simulink model "Simscape_Model"  (R2025b)
settings: Solver=ode15s  StartTime=0.0  StopTime=20  RelTol=1e-3
undefined symbols (not defined in the file): c1, c2, g, k1, k2, kt1, kt2, L1, L2, M1, m1, M2, m2, v1_0, v2_0, X, x1_0, x2_0, Y, Z
libraries: sm_lib x18, nesl_utility x9
settings Model: Creator=Utente  LastModifiedBy=Utente

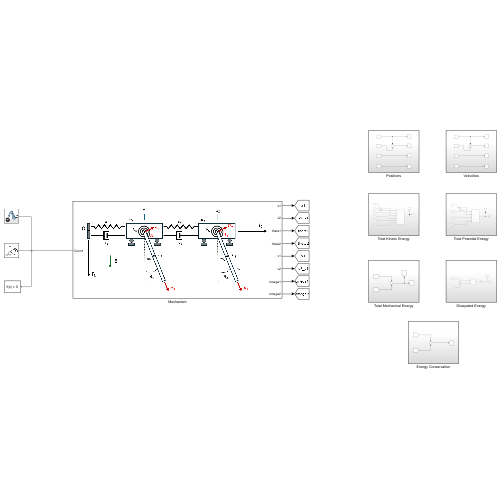
[thumbnail: Simulink's stored preview of the top-level diagram]
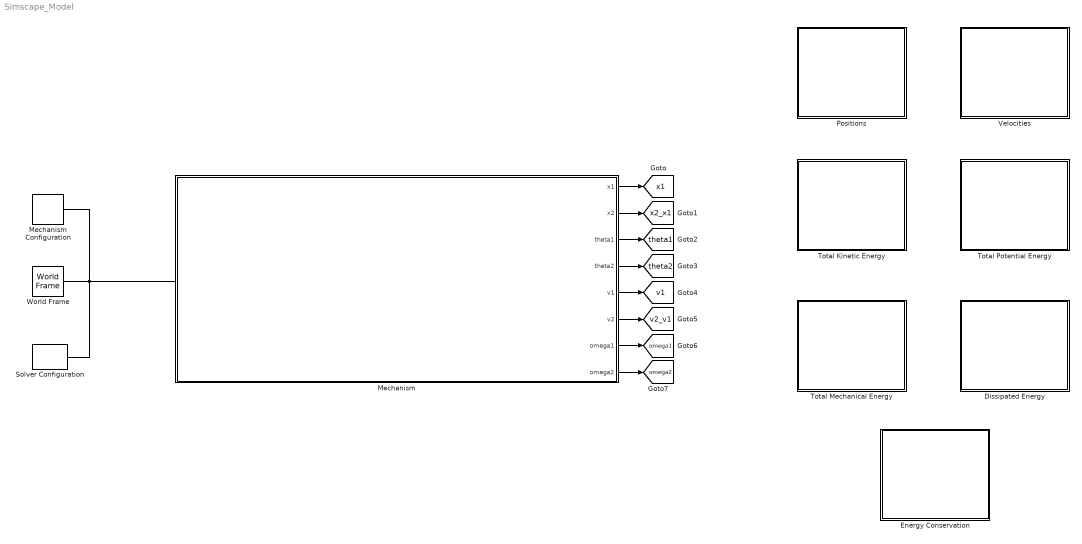
== system Simscape_Model ==
  Dissipated Energy : Subsystem
  Energy Conservation : Subsystem
  Mechanism : Subsystem
      mask Display: image('Frames and Coordinates.png', [20,10,40,10,100,100]);
  Mechanism Configuration : sm_lib/Utilities/Mechanism Configuration  UniformGravity=Constant  GravityVector=[9.80665 0 0]  GravityVectorUnits=m/s^2  LinearizationDelta=0.001  JointModeTransitionNonlinearIterations=2
  Positions : Subsystem
  Solver Configuration : nesl_utility/Solver Configuration  PhysicalDomain=network_engine_domain  SubClassName=solver  LeftPortType=input  RightPortType=generic  Tones=[]  Harmonics=[]  SimulateNoise=off  Profile=off  UseLocalSampling=off  EnableSwitchedLinearOptims=on  FrequencyDomain=off  UseCCode=off  RelTol=0.001  AbsTol=0.001  MinStep=1e-09  ToWorkspace=off  RevertToSquareIcSolve=off  NumHomotopyIterations=100  PhasorMode=off  PhasorModeNumHarmonics=1  ConsistencySolver=NEWTON_XTOL_AFTER_FTOL  IndexReductionMethod=DerivativeReplacement  DoDC=off  ResidualTolerance=1e-09  ConsistencyTolSource=GLOBAL  ConsistencyAbsTol=0.001  ConsistencyRelTol=0.001  ConsistencyTolFactor=0.001  UseLocalSolver=off  LocalSolverChoice=NE_BACKWARD_EULER_ADVANCER  ResolveIndetEquations=on  FunctionEvalNumThread=1  LocalSolverSampleTime=0.001  DoFixedCost=off  MaxNonlinIter=3  MaxModeIter=2  ComputeImpulses=off  ImpulseIterations=2  LinearAlgebra=auto  LinearAlgebraNumThread=0  EquationFormulation=NE_TIME_EF  DelaysMemoryBudget=1024  AutomaticFiltering=on  FilteringTimeConstant=0.001  PartitionStorageMethod=AS_NEEDED  PartitionMemoryBudget=1024  PartitionMethod=ROBUST  MultibodyUseLocalSolver=off  MultibodyLocalSolverChoice=ODE1  MultibodyLocalSolverSampleTime=0.001
  Total Kinetic Energy : Subsystem
  Total Mechanical Energy : Subsystem
  Total Potential Energy : Subsystem
  Velocities : Subsystem
  World Frame : sm_lib/Frames and Transforms/World Frame
  tag scope: omega1=global, omega2=global, theta1=global, theta2=global, v1=global, v2_v1=global, x1=global, x2_x1=global
  wires:
  Mechanism/1(x1) -> [x1]
  Mechanism/2(x2) -> [x2_x1]
  Mechanism/3(theta1) -> [theta1]
  Mechanism/4(theta2) -> [theta2]
  Mechanism/5(v1) -> [v1]
  Mechanism/6(v2) -> [v2_v1]
  Mechanism/7(omega1) -> [omega1]
  Mechanism/8(omega2) -> [omega2]
  connections:
  World Frame/RConn1 -- Solver Configuration/RConn1 -- Mechanism/LConn1 -- Mechanism Configuration/RConn1

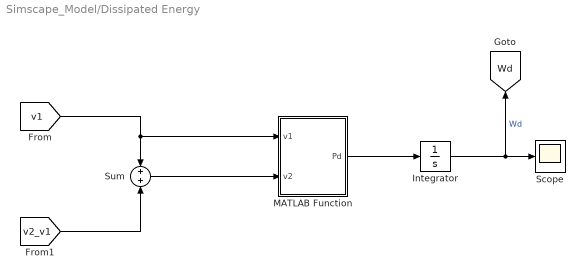
== system Simscape_Model/Dissipated Energy ==
  Integrator : Integrator
  MATLAB Function : MATLAB Function  TreatAsAtomicUnit=on
  Scope : Scope
      settings: ActiveDisplayYMinimum=-0.01761357447503813  ActiveDisplayYMaximum=0.15852217027534321  DataLoggingVariableName=ScopeData11
  Sum : Sum
  tag scope: Wd=global
  wires:
  [v1] -> Sum/1, MATLAB Function/1(v1)
  [v2_v1] -> Sum/2
  Sum/1 -> MATLAB Function/2(v2)
  MATLAB Function/1(Pd) -> Integrator/1
  Integrator/1 -> [Wd], Scope/1  "Wd"

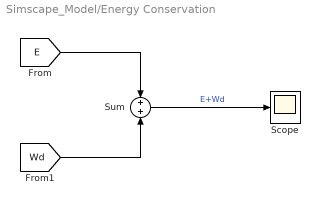
== system Simscape_Model/Energy Conservation ==
  Scope : Scope
      settings: ActiveDisplayYMinimum=0.14074476897436611  ActiveDisplayYMaximum=0.14226416035897949  DataLoggingVariableName=ScopeData12
  Sum : Sum
  wires:
  [E] -> Sum/1
  [Wd] -> Sum/2
  Sum/1 -> Scope/1  "E+Wd"

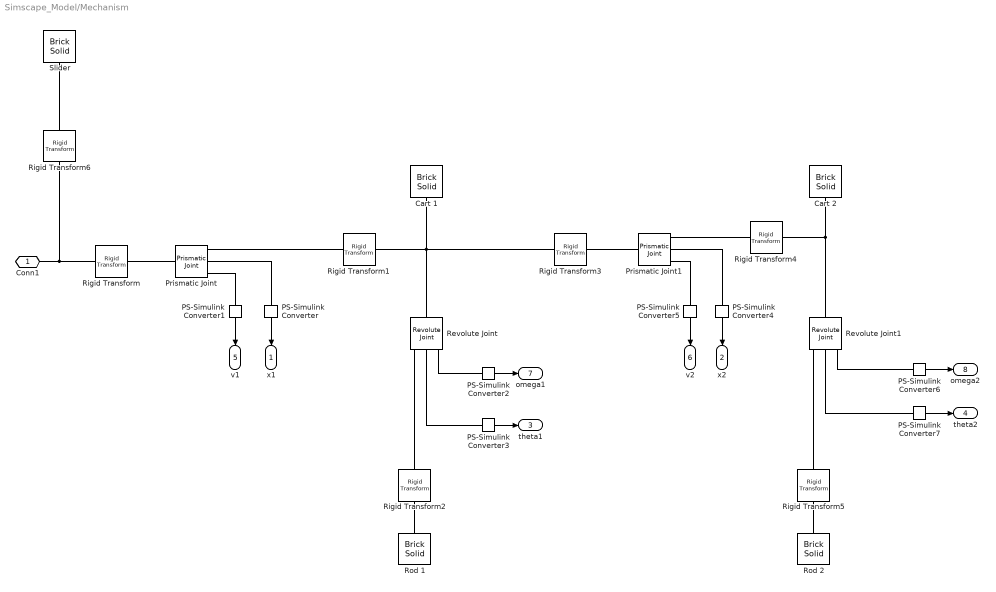
== system Simscape_Model/Mechanism ==
  Cart 1 : sm_lib/Body Elements/Brick Solid  BrickDimensions=[0.1 0.2 0.1]  BrickDimensionsUnits=m  ExportEntireGeometry=off  InertiaType=CalculateFromGeometry  BasedOnType=Mass  Density=1000  DensityUnits=kg/m^3  Mass=M1  MassUnits=kg  CenterOfMass=[0 0 0]  CenterOfMassUnits=m  MomentsOfInertia=[1 1 1]  MomentsOfInertiaUnits=kg*m^2  ProductsOfInertia=[0 0 0]  ProductsOfInertiaUnits=kg*m^2  GraphicType=FromGeometry  MarkerShape=Sphere  MarkerSize=10  GraphicVisPropType=SimpleVisualProperties  GraphicDiffuseColor=[1 0 0]  GraphicOpacity=1  GraphicSpecularColor=[0.5 0.5 0.5 1.0]  GraphicAmbientColor=[0.15 0.15 0.15 1.0]  GraphicEmissiveColor=[0.0 0.0 0.0 1.0]  GraphicShininess=75  DoExposeReferenceFrame=on  SerializedFrames=<Frames/>
  Cart 2 : sm_lib/Body Elements/Brick Solid  BrickDimensions=[0.1 0.2 0.1]  BrickDimensionsUnits=m  ExportEntireGeometry=off  InertiaType=CalculateFromGeometry  BasedOnType=Mass  Density=1000  DensityUnits=kg/m^3  Mass=M2  MassUnits=kg  CenterOfMass=[0 0 0]  CenterOfMassUnits=m  MomentsOfInertia=[1 1 1]  MomentsOfInertiaUnits=kg*m^2  ProductsOfInertia=[0 0 0]  ProductsOfInertiaUnits=kg*m^2  GraphicType=FromGeometry  MarkerShape=Sphere  MarkerSize=10  GraphicVisPropType=SimpleVisualProperties  GraphicDiffuseColor=[1 0 0]  GraphicOpacity=1  GraphicSpecularColor=[0.5 0.5 0.5 1.0]  GraphicAmbientColor=[0.15 0.15 0.15 1.0]  GraphicEmissiveColor=[0.0 0.0 0.0 1.0]  GraphicShininess=75  DoExposeReferenceFrame=on  SerializedFrames=<Frames/>
  PS-Simulink Converter{,1..7} (8 alike) : nesl_utility/PS-Simulink Converter  PhysicalDomain=network_engine_domain  SubClassName=ps_output  LeftPortType=input  RightPortType=output  PseudoPeriodic=off  Frequencies=[]  VectorFormat=inherit  Unit=inherit  AffineConversion=off
  Prismatic Joint : sm_lib/Joints/Prismatic Joint  JointMode=Normal  CompositeWrenchDir=FollowerOnBase  CompositeWrenchFrame=BaseFrame  SenseConstraintForce=off  SenseConstraintTorque=off  SenseTotalForce=off  SenseTotalTorque=off  PositionTargetSpecify=on  PositionTargetPriority=High  PositionTargetValue=x1_0  PositionTargetValueUnits=m  VelocityTargetSpecify=on  VelocityTargetPriority=High  VelocityTargetValue=v1_0  VelocityTargetValueUnits=m/s  EquilibriumPosition=0  EquilibriumPositionUnits=m  SpringStiffness=k1  SpringStiffnessUnits=N/m  DampingCoefficient=c1  DampingCoefficientUnits=N/(m/s)  LowerLimitSpecify=off  LowerLimitBound=-1  LowerLimitBoundUnits=m  LowerLimitStiffness=1e6  LowerLimitStiffnessUnits=N/m  LowerLimitDamping=1e3  LowerLimitDampingUnits=N/(m/s)  LowerLimitTransitionRegionWidth=1e-4  LowerLimitTransitionRegionWidthUnits=m  UpperLimitSpecify=off  UpperLimitBound=1  UpperLimitBoundUnits=m  UpperLimitStiffness=1e6  UpperLimitStiffnessUnits=N/m  UpperLimitDamping=1e3  UpperLimitDampingUnits=N/(m/s)  UpperLimitTransitionRegionWidth=1e-4  UpperLimitTransitionRegionWidthUnits=m  TorqueActuationMode=NoTorque  MotionActuationMode=ComputedMotion  SensePosition=on  SenseVelocity=on  SenseAcceleration=off  SenseTorqueForce=off  SenseLowerLimitTorqueForce=off  SenseUpperLimitTorqueForce=off
  Prismatic Joint1 : sm_lib/Joints/Prismatic Joint  JointMode=Normal  CompositeWrenchDir=FollowerOnBase  CompositeWrenchFrame=BaseFrame  SenseConstraintForce=off  SenseConstraintTorque=off  SenseTotalForce=off  SenseTotalTorque=off  PositionTargetSpecify=on  PositionTargetPriority=High  PositionTargetValue=x2_0-x1_0  PositionTargetValueUnits=m  VelocityTargetSpecify=on  VelocityTargetPriority=High  VelocityTargetValue=v2_0-v1_0  VelocityTargetValueUnits=m/s  EquilibriumPosition=0  EquilibriumPositionUnits=m  SpringStiffness=k2  SpringStiffnessUnits=N/m  DampingCoefficient=c2  DampingCoefficientUnits=N/(m/s)  LowerLimitSpecify=off  LowerLimitBound=-1  LowerLimitBoundUnits=m  LowerLimitStiffness=1e6  LowerLimitStiffnessUnits=N/m  LowerLimitDamping=1e3  LowerLimitDampingUnits=N/(m/s)  LowerLimitTransitionRegionWidth=1e-4  LowerLimitTransitionRegionWidthUnits=m  UpperLimitSpecify=off  UpperLimitBound=1  UpperLimitBoundUnits=m  UpperLimitStiffness=1e6  UpperLimitStiffnessUnits=N/m  UpperLimitDamping=1e3  UpperLimitDampingUnits=N/(m/s)  UpperLimitTransitionRegionWidth=1e-4  UpperLimitTransitionRegionWidthUnits=m  TorqueActuationMode=NoTorque  MotionActuationMode=ComputedMotion  SensePosition=on  SenseVelocity=on  SenseAcceleration=off  SenseTorqueForce=off  SenseLowerLimitTorqueForce=off  SenseUpperLimitTorqueForce=off
  Revolute Joint : sm_lib/Joints/Revolute Joint  JointMode=Normal  CompositeWrenchDir=FollowerOnBase  CompositeWrenchFrame=BaseFrame  SenseConstraintForce=off  SenseConstraintTorque=off  SenseTotalForce=off  SenseTotalTorque=off  PositionTargetSpecify=on  PositionTargetPriority=High  PositionTargetValue=theta1_0  PositionTargetValueUnits=rad  VelocityTargetSpecify=on  VelocityTargetPriority=High  VelocityTargetValue=omega1_0  VelocityTargetValueUnits=rad/s  EquilibriumPosition=0  EquilibriumPositionUnits=deg  SpringStiffness=kt1  SpringStiffnessUnits=N*m/rad  DampingCoefficient=0  DampingCoefficientUnits=N*m/(deg/s)  LowerLimitSpecify=off  LowerLimitBound=-90  LowerLimitBoundUnits=deg  LowerLimitStiffness=1e4  LowerLimitStiffnessUnits=N*m/deg  LowerLimitDamping=10  LowerLimitDampingUnits=N*m/(deg/s)  LowerLimitTransitionRegionWidth=0.1  LowerLimitTransitionRegionWidthUnits=deg  UpperLimitSpecify=off  UpperLimitBound=90  UpperLimitBoundUnits=deg  UpperLimitStiffness=1e4  UpperLimitStiffnessUnits=N*m/deg  UpperLimitDamping=10  UpperLimitDampingUnits=N*m/(deg/s)  UpperLimitTransitionRegionWidth=0.1  UpperLimitTransitionRegionWidthUnits=deg  TorqueActuationMode=NoTorque  MotionActuationMode=ComputedMotion  SensePosition=on  SenseVelocity=on  SenseAcceleration=off  SenseTorqueForce=off  SenseLowerLimitTorqueForce=off  SenseUpperLimitTorqueForce=off
  Revolute Joint1 : sm_lib/Joints/Revolute Joint  JointMode=Normal  CompositeWrenchDir=FollowerOnBase  CompositeWrenchFrame=BaseFrame  SenseConstraintForce=off  SenseConstraintTorque=off  SenseTotalForce=off  SenseTotalTorque=off  PositionTargetSpecify=on  PositionTargetPriority=High  PositionTargetValue=theta2_0  PositionTargetValueUnits=rad  VelocityTargetSpecify=on  VelocityTargetPriority=High  VelocityTargetValue=omega2_0  VelocityTargetValueUnits=rad/s  EquilibriumPosition=0  EquilibriumPositionUnits=deg  SpringStiffness=kt2  SpringStiffnessUnits=N*m/rad  DampingCoefficient=0  DampingCoefficientUnits=N*m/(deg/s)  LowerLimitSpecify=off  LowerLimitBound=-90  LowerLimitBoundUnits=deg  LowerLimitStiffness=1e4  LowerLimitStiffnessUnits=N*m/deg  LowerLimitDamping=10  LowerLimitDampingUnits=N*m/(deg/s)  LowerLimitTransitionRegionWidth=0.1  LowerLimitTransitionRegionWidthUnits=deg  UpperLimitSpecify=off  UpperLimitBound=90  UpperLimitBoundUnits=deg  UpperLimitStiffness=1e4  UpperLimitStiffnessUnits=N*m/deg  UpperLimitDamping=10  UpperLimitDampingUnits=N*m/(deg/s)  UpperLimitTransitionRegionWidth=0.1  UpperLimitTransitionRegionWidthUnits=deg  TorqueActuationMode=NoTorque  MotionActuationMode=ComputedMotion  SensePosition=on  SenseVelocity=on  SenseAcceleration=off  SenseTorqueForce=off  SenseLowerLimitTorqueForce=off  SenseUpperLimitTorqueForce=off
  Rigid Transform : sm_lib/Frames and Transforms/Rigid Transform  RotationMethod=StandardAxis  FollAlignAxisA=+X  BaseAlignAxisA=+Y  FollAlignAxisB=+Y  BaseAlignAxisB=+Z  RotationStandardAxis=+X  RotationAngle=-90  RotationAngleUnits=deg  RotationArbitraryAxis=[0 0 1]  RotationSequenceAxes=FollowerAxes  RotationSequence=XYX  RotationSequenceAngles=[0 0 0]  RotationSequenceAnglesUnits=deg  RotationMatrix=[1 0 0;0 1 0;0 0 1]  Quaternion=[1 0 0 0]  TranslationMethod=None  TranslationCartesianOffset=[0 0 0]  TranslationCartesianOffsetUnits=m  TranslationStandardAxis=+Z  TranslationStandardOffset=0  TranslationStandardOffsetUnits=m  TranslationROffset=0  TranslationROffsetUnits=m  TranslationThetaOffset=0  TranslationThetaOffsetUnits=deg  TranslationZOffset=0  TranslationZOffsetUnits=m
  Rigid Transform1 : sm_lib/Frames and Transforms/Rigid Transform  RotationMethod=StandardAxis  FollAlignAxisA=+X  BaseAlignAxisA=+Y  FollAlignAxisB=+Y  BaseAlignAxisB=+Z  RotationStandardAxis=+X  RotationAngle=90  RotationAngleUnits=deg  RotationArbitraryAxis=[0 0 1]  RotationSequenceAxes=FollowerAxes  RotationSequence=XYX  RotationSequenceAngles=[0 0 0]  RotationSequenceAnglesUnits=deg  RotationMatrix=[1 0 0;0 1 0;0 0 1]  Quaternion=[1 0 0 0]  TranslationMethod=None  TranslationCartesianOffset=[0 0 0]  TranslationCartesianOffsetUnits=m  TranslationStandardAxis=+Z  TranslationStandardOffset=0  TranslationStandardOffsetUnits=m  TranslationROffset=0  TranslationROffsetUnits=m  TranslationThetaOffset=0  TranslationThetaOffsetUnits=deg  TranslationZOffset=0  TranslationZOffsetUnits=m
  Rigid Transform2 : sm_lib/Frames and Transforms/Rigid Transform  RotationMethod=None  FollAlignAxisA=+X  BaseAlignAxisA=+Y  FollAlignAxisB=+Y  BaseAlignAxisB=+Z  RotationStandardAxis=+Z  RotationAngle=0  RotationAngleUnits=deg  RotationArbitraryAxis=[0 0 1]  RotationSequenceAxes=FollowerAxes  RotationSequence=XYX  RotationSequenceAngles=[0 0 0]  RotationSequenceAnglesUnits=deg  RotationMatrix=[1 0 0;0 1 0;0 0 1]  Quaternion=[1 0 0 0]  TranslationMethod=Cartesian  TranslationCartesianOffset=[L1/2 0 0]  TranslationCartesianOffsetUnits=m  TranslationStandardAxis=+Z  TranslationStandardOffset=0  TranslationStandardOffsetUnits=m  TranslationROffset=0  TranslationROffsetUnits=m  TranslationThetaOffset=0  TranslationThetaOffsetUnits=deg  TranslationZOffset=0  TranslationZOffsetUnits=m
  Rigid Transform3 : sm_lib/Frames and Transforms/Rigid Transform  RotationMethod=StandardAxis  FollAlignAxisA=+X  BaseAlignAxisA=+Y  FollAlignAxisB=+Y  BaseAlignAxisB=+Z  RotationStandardAxis=+X  RotationAngle=-90  RotationAngleUnits=deg  RotationArbitraryAxis=[0 0 1]  RotationSequenceAxes=FollowerAxes  RotationSequence=XYX  RotationSequenceAngles=[0 0 0]  RotationSequenceAnglesUnits=deg  RotationMatrix=[1 0 0;0 1 0;0 0 1]  Quaternion=[1 0 0 0]  TranslationMethod=Cartesian  TranslationCartesianOffset=[0 0.5 0]  TranslationCartesianOffsetUnits=m  TranslationStandardAxis=+Z  TranslationStandardOffset=0  TranslationStandardOffsetUnits=m  TranslationROffset=0  TranslationROffsetUnits=m  TranslationThetaOffset=0  TranslationThetaOffsetUnits=deg  TranslationZOffset=0  TranslationZOffsetUnits=m
  Rigid Transform4 : sm_lib/Frames and Transforms/Rigid Transform  RotationMethod=StandardAxis  FollAlignAxisA=+X  BaseAlignAxisA=+Y  FollAlignAxisB=+Y  BaseAlignAxisB=+Z  RotationStandardAxis=+X  RotationAngle=90  RotationAngleUnits=deg  RotationArbitraryAxis=[0 0 1]  RotationSequenceAxes=FollowerAxes  RotationSequence=XYX  RotationSequenceAngles=[0 0 0]  RotationSequenceAnglesUnits=deg  RotationMatrix=[1 0 0;0 1 0;0 0 1]  Quaternion=[1 0 0 0]  TranslationMethod=None  TranslationCartesianOffset=[0 0 0]  TranslationCartesianOffsetUnits=m  TranslationStandardAxis=+Z  TranslationStandardOffset=0  TranslationStandardOffsetUnits=m  TranslationROffset=0  TranslationROffsetUnits=m  TranslationThetaOffset=0  TranslationThetaOffsetUnits=deg  TranslationZOffset=0  TranslationZOffsetUnits=m
  Rigid Transform5 : sm_lib/Frames and Transforms/Rigid Transform  RotationMethod=None  FollAlignAxisA=+X  BaseAlignAxisA=+Y  FollAlignAxisB=+Y  BaseAlignAxisB=+Z  RotationStandardAxis=+Z  RotationAngle=0  RotationAngleUnits=deg  RotationArbitraryAxis=[0 0 1]  RotationSequenceAxes=FollowerAxes  RotationSequence=XYX  RotationSequenceAngles=[0 0 0]  RotationSequenceAnglesUnits=deg  RotationMatrix=[1 0 0;0 1 0;0 0 1]  Quaternion=[1 0 0 0]  TranslationMethod=Cartesian  TranslationCartesianOffset=[L2/2 0 0]  TranslationCartesianOffsetUnits=m  TranslationStandardAxis=+Z  TranslationStandardOffset=0  TranslationStandardOffsetUnits=m  TranslationROffset=0  TranslationROffsetUnits=m  TranslationThetaOffset=0  TranslationThetaOffsetUnits=deg  TranslationZOffset=0  TranslationZOffsetUnits=m
  Rigid Transform6 : sm_lib/Frames and Transforms/Rigid Transform  RotationMethod=None  FollAlignAxisA=+X  BaseAlignAxisA=+Y  FollAlignAxisB=+Y  BaseAlignAxisB=+Z  RotationStandardAxis=+Z  RotationAngle=0  RotationAngleUnits=deg  RotationArbitraryAxis=[0 0 1]  RotationSequenceAxes=FollowerAxes  RotationSequence=XYX  RotationSequenceAngles=[0 0 0]  RotationSequenceAnglesUnits=deg  RotationMatrix=[1 0 0;0 1 0;0 0 1]  Quaternion=[1 0 0 0]  TranslationMethod=Cartesian  TranslationCartesianOffset=[0 0.25 0]  TranslationCartesianOffsetUnits=m  TranslationStandardAxis=+Z  TranslationStandardOffset=0  TranslationStandardOffsetUnits=m  TranslationROffset=0  TranslationROffsetUnits=m  TranslationThetaOffset=0  TranslationThetaOffsetUnits=deg  TranslationZOffset=0  TranslationZOffsetUnits=m
  Rod 1 : sm_lib/Body Elements/Brick Solid  BrickDimensions=[L1 0.01 0.01]  BrickDimensionsUnits=m  ExportEntireGeometry=off  InertiaType=CalculateFromGeometry  BasedOnType=Mass  Density=1000  DensityUnits=kg/m^3  Mass=m1  MassUnits=kg  CenterOfMass=[0 0 0]  CenterOfMassUnits=m  MomentsOfInertia=[1 1 1]  MomentsOfInertiaUnits=kg*m^2  ProductsOfInertia=[0 0 0]  ProductsOfInertiaUnits=kg*m^2  GraphicType=FromGeometry  MarkerShape=Sphere  MarkerSize=10  GraphicVisPropType=SimpleVisualProperties  GraphicDiffuseColor=[0.5 0.5 0.5]  GraphicOpacity=1  GraphicSpecularColor=[0.5 0.5 0.5 1.0]  GraphicAmbientColor=[0.15 0.15 0.15 1.0]  GraphicEmissiveColor=[0.0 0.0 0.0 1.0]  GraphicShininess=75  DoExposeReferenceFrame=on  SerializedFrames=<Frames/>
  Rod 2 : sm_lib/Body Elements/Brick Solid  BrickDimensions=[L2 0.01 0.01]  BrickDimensionsUnits=m  ExportEntireGeometry=off  InertiaType=CalculateFromGeometry  BasedOnType=Mass  Density=1000  DensityUnits=kg/m^3  Mass=m2  MassUnits=kg  CenterOfMass=[0 0 0]  CenterOfMassUnits=m  MomentsOfInertia=[1 1 1]  MomentsOfInertiaUnits=kg*m^2  ProductsOfInertia=[0 0 0]  ProductsOfInertiaUnits=kg*m^2  GraphicType=FromGeometry  MarkerShape=Sphere  MarkerSize=10  GraphicVisPropType=SimpleVisualProperties  GraphicDiffuseColor=[0.5 0.5 0.5]  GraphicOpacity=1  GraphicSpecularColor=[0.5 0.5 0.5 1.0]  GraphicAmbientColor=[0.15 0.15 0.15 1.0]  GraphicEmissiveColor=[0.0 0.0 0.0 1.0]  GraphicShininess=75  DoExposeReferenceFrame=on  SerializedFrames=<Frames/>
  Slider : sm_lib/Body Elements/Brick Solid  BrickDimensions=[0.01 1.0 0.01]  BrickDimensionsUnits=m  ExportEntireGeometry=off  InertiaType=CalculateFromGeometry  BasedOnType=Mass  Density=1000  DensityUnits=kg/m^3  Mass=1e-6  MassUnits=kg  CenterOfMass=[0 0 0]  CenterOfMassUnits=m  MomentsOfInertia=[1 1 1]  MomentsOfInertiaUnits=kg*m^2  ProductsOfInertia=[0 0 0]  ProductsOfInertiaUnits=kg*m^2  GraphicType=FromGeometry  MarkerShape=Sphere  MarkerSize=10  GraphicVisPropType=SimpleVisualProperties  GraphicDiffuseColor=[0 0 0]  GraphicOpacity=1  GraphicSpecularColor=[0.5 0.5 0.5 1.0]  GraphicAmbientColor=[0.15 0.15 0.15 1.0]  GraphicEmissiveColor=[0.0 0.0 0.0 1.0]  GraphicShininess=75  DoExposeReferenceFrame=on  SerializedFrames=<Frames/>
  Conn1 : PMIOPort  Side=Left
  x1 : Outport
  x2 : Outport  Port=2
  theta1 : Outport  Port=3
  theta2 : Outport  Port=4
  v1 : Outport  Port=5
  v2 : Outport  Port=6
  omega1 : Outport  Port=7
  omega2 : Outport  Port=8
  wires:
  PS-Simulink Converter1/1 -> v1/1
  PS-Simulink Converter/1 -> x1/1
  PS-Simulink Converter2/1 -> omega1/1
  PS-Simulink Converter3/1 -> theta1/1
  PS-Simulink Converter5/1 -> v2/1
  PS-Simulink Converter4/1 -> x2/1
  PS-Simulink Converter6/1 -> omega2/1
  PS-Simulink Converter7/1 -> theta2/1
  connections:
  Rigid Transform2/LConn1 -- Revolute Joint/RConn1
  Rigid Transform1/LConn1 -- Prismatic Joint/RConn1
  Rigid Transform/LConn1 -- Rigid Transform6/LConn1 -- Conn1/RConn1
  Revolute Joint/LConn1 -- Rigid Transform1/RConn1 -- Cart 1/RConn1 -- Rigid Transform3/LConn1
  PS-Simulink Converter1/LConn1 -- Prismatic Joint/RConn3
  Prismatic Joint/LConn1 -- Rigid Transform/RConn1
  Rigid Transform4/RConn1 -- Revolute Joint1/LConn1 -- Cart 2/RConn1
  Rigid Transform5/LConn1 -- Revolute Joint1/RConn1
  Rod 1/RConn1 -- Rigid Transform2/RConn1
  Rod 2/RConn1 -- Rigid Transform5/RConn1
  Prismatic Joint1/LConn1 -- Rigid Transform3/RConn1
  Prismatic Joint/RConn2 -- PS-Simulink Converter/LConn1
  Rigid Transform4/LConn1 -- Prismatic Joint1/RConn1
  Revolute Joint/RConn3 -- PS-Simulink Converter2/LConn1
  PS-Simulink Converter3/LConn1 -- Revolute Joint/RConn2
  Prismatic Joint1/RConn2 -- PS-Simulink Converter4/LConn1
  Prismatic Joint1/RConn3 -- PS-Simulink Converter5/LConn1
  Revolute Joint1/RConn3 -- PS-Simulink Converter6/LConn1
  Revolute Joint1/RConn2 -- PS-Simulink Converter7/LConn1
  Rigid Transform6/RConn1 -- Slider/RConn1

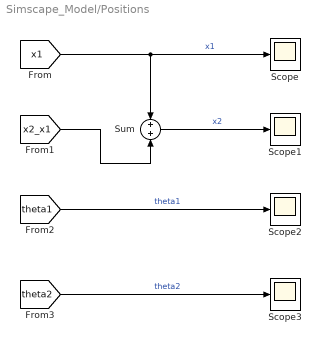
== system Simscape_Model/Positions ==
  Scope{,1..3} (4 alike) : Scope
      Scope settings: ActiveDisplayYMinimum=-0.047917640365799409  ActiveDisplayYMaximum=0.031258763292194694
      Scope1 settings: ActiveDisplayYMinimum=-0.020428735704603108  ActiveDisplayYMaximum=0.046714303967178121
      Scope2 settings: ActiveDisplayYMinimum=-0.43106744677904457  ActiveDisplayYMaximum=0.39952098178738554  DataLoggingVariableName=ScopeData2
      Scope3 settings: ActiveDisplayYMinimum=-0.27459437543170317  ActiveDisplayYMaximum=0.26599766787507068  DataLoggingVariableName=ScopeData3
  Sum : Sum
  wires:
  [x1] -> Sum/1, Scope/1  "x1"
  [x2_x1] -> Sum/2
  Sum/1 -> Scope1/1  "x2"
  [theta1] -> Scope2/1  "theta1"
  [theta2] -> Scope3/1  "theta2"

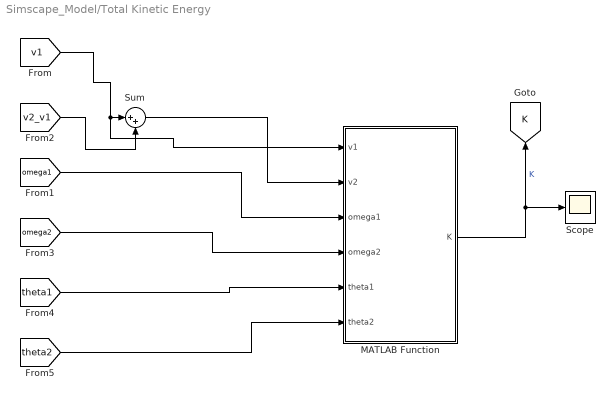
== system Simscape_Model/Total Kinetic Energy ==
  MATLAB Function : MATLAB Function  TreatAsAtomicUnit=on
  Scope : Scope
      settings: ActiveDisplayYMinimum=-0.010342980181834159  ActiveDisplayYMaximum=0.093086821636507444  DataLoggingVariableName=ScopeData8
  Sum : Sum  Inputs=|++
  tag scope: K=global
  wires:
  [v1] -> Sum/1, MATLAB Function/1(v1)
  [v2_v1] -> Sum/2
  [omega1] -> MATLAB Function/3(omega1)
  [omega2] -> MATLAB Function/4(omega2)
  [theta1] -> MATLAB Function/5(theta1)
  [theta2] -> MATLAB Function/6(theta2)
  MATLAB Function/1(K) -> [K], Scope/1  "K"
  Sum/1 -> MATLAB Function/2(v2)

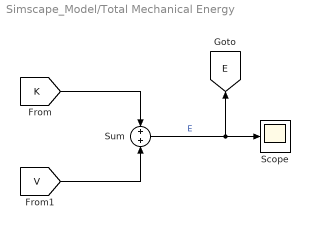
== system Simscape_Model/Total Mechanical Energy ==
  Scope : Scope
      settings: ActiveDisplayYMinimum=-0.01774516632283183  ActiveDisplayYMaximum=0.15975435828410445  DataLoggingVariableName=ScopeData10
  Sum : Sum
  tag scope: E=global
  wires:
  [K] -> Sum/1
  [V] -> Sum/2
  Sum/1 -> [E], Scope/1  "E"

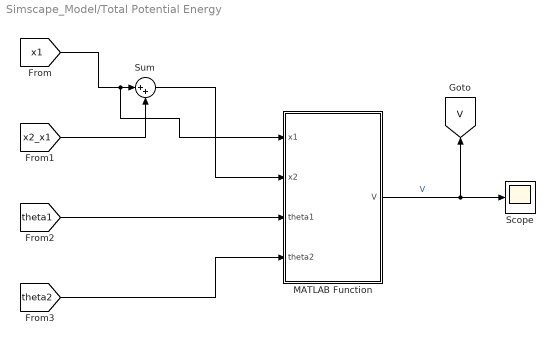
== system Simscape_Model/Total Potential Energy ==
  MATLAB Function : MATLAB Function  TreatAsAtomicUnit=on
  Scope : Scope
      settings: ActiveDisplayYMinimum=-0.017750209666827461  ActiveDisplayYMaximum=0.15975491865565952  DataLoggingVariableName=ScopeData9
  Sum : Sum  Inputs=|++
  tag scope: V=global
  wires:
  [x1] -> MATLAB Function/1(x1), Sum/1
  [x2_x1] -> Sum/2
  Sum/1 -> MATLAB Function/2(x2)
  [theta1] -> MATLAB Function/3(theta1)
  [theta2] -> MATLAB Function/4(theta2)
  MATLAB Function/1(V) -> Scope/1, [V]  "V"

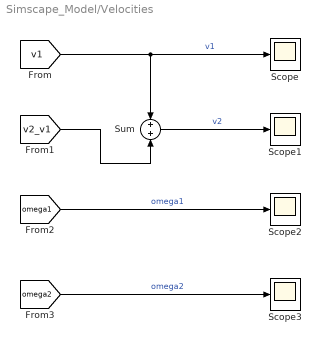
== system Simscape_Model/Velocities ==
  Scope{,1..3} (4 alike) : Scope
      Scope settings: ActiveDisplayYMinimum=-0.20065998758591308  ActiveDisplayYMaximum=0.36407695728293882  DataLoggingVariableName=ScopeData4
      Scope1 settings: ActiveDisplayYMinimum=-0.26382490873400122  ActiveDisplayYMaximum=0.17109213595692183  DataLoggingVariableName=ScopeData5
      Scope2 settings: ActiveDisplayYMinimum=-3.4696160274432875  ActiveDisplayYMaximum=3.3596136306059776  DataLoggingVariableName=ScopeData6
      Scope3 settings: ActiveDisplayYMinimum=-2.47984605497847  ActiveDisplayYMaximum=2.6306663373988557  DataLoggingVariableName=ScopeData7
  Sum : Sum
  wires:
  [v2_v1] -> Sum/2
  Sum/1 -> Scope1/1  "v2"
  [omega2] -> Scope3/1  "omega2"
  [omega1] -> Scope2/1  "omega1"
  [v1] -> Sum/1, Scope/1  "v1"

== matlab function Simscape_Model/Total Potential Energy/MATLAB Function ==
  data: x1 input; V output; x2 input; theta1 input; theta2 input; m1 parameter; m2 parameter; L1 parameter; L2 parameter; k1 parameter; k2 parameter; kt1 parameter; kt2 parameter; g parameter
function V = fcn(x1, x2, theta1, theta2, m1, m2, L1, L2, k1, k2, kt1, kt2, g)

% Gravitational potential energy
Vg = m1*g*L1/2*(1 - cos(theta1)) + m2*g*L2/2*(1 - cos(theta2));

% Elastic potential energy
Ve = 0.5*k1*x1^2 + 0.5*k2*(x2 - x1)^2 + 0.5*kt1*theta1^2 + 0.5*kt2*theta2^2;

V = Vg + Ve;

end

== matlab function Simscape_Model/Total Kinetic Energy/MATLAB Function ==
  data: v1 input; v2 input; omega1 input; omega2 input; theta1 input; K output; theta2 input; M1 parameter; M2 parameter; L1 parameter; L2 parameter; m1 parameter; m2 parameter
function K = fcn(v1, v2, omega1, omega2, theta1, theta2, M1, M2, L1, L2, m1, m2)

K_carts = 0.5*M1*v1^2 + 0.5*M2*v2^2;

K_rod1 = 0.5*m1*v1^2 + 0.5*(m1*L1^2/3)*omega1^2 + 0.5*m1*L1*cos(theta1)*v1*omega1;

K_rod2 = 0.5*m2*v2^2 + 0.5*(m2*L2^2/3)*omega2^2 + 0.5*m2*L2*cos(theta2)*v2*omega2;

K = K_carts + K_rod1 + K_rod2;

end

== matlab function Simscape_Model/Dissipated Energy/MATLAB Function ==
  data: v1 input; Pd output; v2 input; c1 parameter; c2 parameter
function Pd = fcn(v1, v2, c1, c2)

Pd = c1*v1^2 + c2*(v2 - v1)^2;

end
